simulink model "FSI_1DOF_Simscape"  (R2024a)
settings: Solver=FixedStepAuto  StartTime=0.0  StopTime=5  FixedStep=1e-4  MaxStep=1e-5  MinStep=1e-5  RelTol=1e-6  EnableMultiTasking=on
InitFcn:
  | FSI_1DOF_Simscape_init
values from neighbouring files (symbols this model uses):
  b = (2*m*omega_0)/(2*Q)    (= 3.14159265359)    [FSI_1DOF_Simscape_init.m]
  bias_exc = 0    [FSI_1DOF_Simscape_init.m]
  F_exc = 10    [FSI_1DOF_Simscape_init.m]
  omega_exc = 2*pi*freq_exc    (= 62.8318530718)    [FSI_1DOF_Simscape_init.m]
  phase_exc = 0    [FSI_1DOF_Simscape_init.m]
  t_step = 1e-2    (= 0.01)    [FSI_1DOF_Simscape_init.m]
libraries: fl_lib x8, nesl_utility x4
settings Model: Creator=FilipKsica  LastModifiedBy=144901
settings SolverCC: InitialStep=1e-5  AlgebraicLoopSolver=TrustRegion
settings DataIOCC: LimitDataPoints=on  ReturnWorkspaceOutputs=off
settings OptimizationCC: LifeSpan=inf
settings DebuggingCC: UnconnectedInputMsg=warning  UnconnectedOutputMsg=warning  UnconnectedLineMsg=warning  AllowSymbolicDim=off  SFUnexpectedBacktrackingDiag=warning  SFNoUnconditionalDefaultTransitionDiag=warning  SFExecutionAtInitializationDiag=none  ArithmeticOperatorsInVariantConditions=warning
settings ModelReferenceCC: EnableRefExpFcnMdlSchedulingChecks=on  PropagateSignalLabelsOutOfModel=off
settings SFSimCC: SimUseLocalCustomCode=off  CustomCodeUndefinedFunction=UseInterfaceOnly
settings RTWCC: RTWUseLocalCustomCode=off  GPUComputeCapability=3.5  DLArmComputeVersion=19.05
settings CodeAppCC: StateflowObjectComments=on
settings GRTTargetCC: TargetLangStandard=C89/C90 (ANSI)
settings ConfigComp: CovMetricSettings=dw  CovSaveCumulativeToWorkspaceVar=on  CovSaveSingleToWorkspaceVar=on  CovExternalEMLEnable=off
settings SimscapeCC: SimscapeNormalizeSystem=off

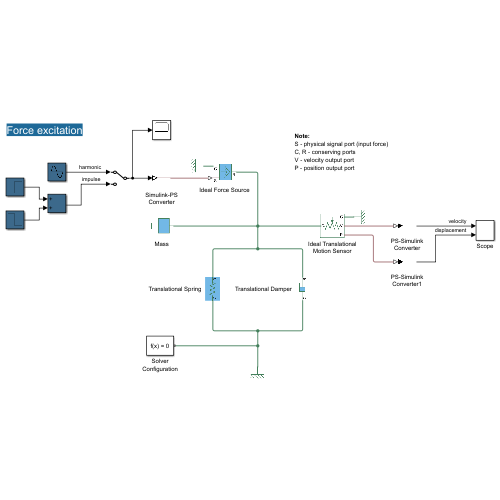
[thumbnail: Simulink's stored preview of the top-level diagram]
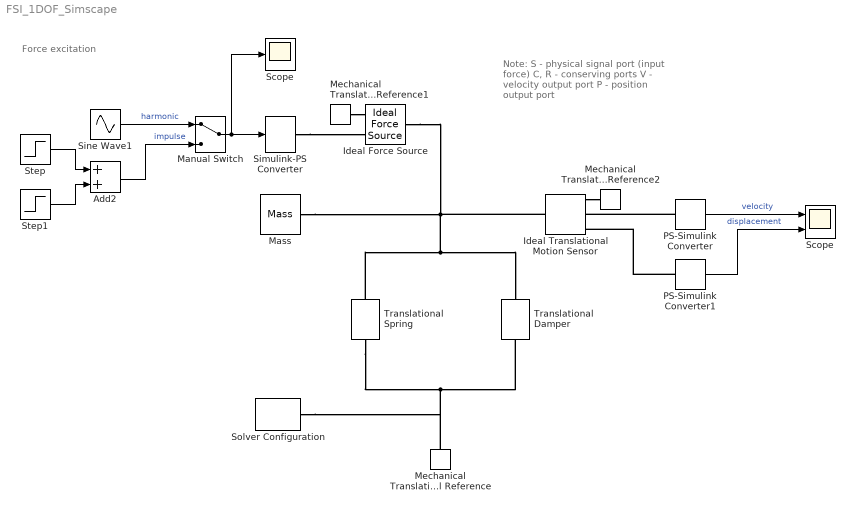
== system FSI_1DOF_Simscape ==
  note: Note:
      | S - physical signal port (input force)
      | C, R - conserving ports
      | V - velocity output port
      | P - position output port
  note: Force excitation
  Add2 : Sum
  Ideal Force Source : fl_lib/Mechanical/Mechanical Sources/Ideal Force Source
  Ideal Translational Motion Sensor : fl_lib/Mechanical/Mechanical Sensors/Ideal Translational Motion Sensor  reference=foundation.enum.MeasurementReference.difference  acceleration_port=false  velocity_port=true  position_port=true  offset=0 m
  Manual Switch : ManualSwitch
  Mass : fl_lib/Mechanical/Translational Elements/Mass  mass=m kg  num_ports=foundation.enum.numPorts2.one  v_specify=off  v_priority=None  v=0 m/s  v_nominal_specify=off  v_nominal_value=1  v_nominal_unit=m/s  f_specify=off  f_priority=None  f=0 N  f_nominal_specify=off  f_nominal_value=1  f_nominal_unit=N
  Mechanical Translational Reference : fl_lib/Mechanical/Translational Elements/Mechanical Translational Reference
  Mechanical Translational Reference1 : fl_lib/Mechanical/Translational Elements/Mechanical Translational Reference
  Mechanical Translational Reference2 : fl_lib/Mechanical/Translational Elements/Mechanical Translational Reference
  PS-Simulink Converter : nesl_utility/PS-Simulink Converter  PhysicalDomain=network_engine_domain  SubClassName=ps_output  LeftPortType=input  RightPortType=output  PseudoPeriodic=off  Frequencies=[]  VectorFormat=1-D array  Unit=1  AffineConversion=off
  PS-Simulink Converter1 : nesl_utility/PS-Simulink Converter  PhysicalDomain=network_engine_domain  SubClassName=ps_output  LeftPortType=input  RightPortType=output  PseudoPeriodic=off  Frequencies=[]  VectorFormat=1-D array  Unit=1  AffineConversion=off
  Scope : Scope
  "Scope " : Scope  NumInputPorts=2
  Simulink-PS Converter : nesl_utility/Simulink-PS Converter  PhysicalDomain=network_engine_domain  SubClassName=ps_input  LeftPortType=input  RightPortType=output  PseudoPeriodic=off  Frequencies=[]  NoiseDistribution=none  NoiseParameters=[]  Unit=1  AffineConversion=off  FilteringAndDerivatives=zero  SimscapeFilterOrder=1  InputFilterTimeConstant=0.001  UdotUserProvided=1
  Sine Wave1 : Sin  Amplitude=F_exc  Bias=bias_exc  Frequency=omega_exc  Phase=phase_exc  SampleTime=0
  Solver Configuration : nesl_utility/Solver Configuration  PhysicalDomain=network_engine_domain  SubClassName=solver  LeftPortType=input  RightPortType=generic  Tones=[]  Harmonics=[]  SimulateNoise=off  Profile=off  UseLocalSampling=off  EnableSwitchedLinearOptims=on  FrequencyDomain=off  UseCCode=off  RelTol=0.001  AbsTol=1e-06  MinStep=1e-09  ToWorkspace=off  RevertToSquareIcSolve=off  NumHomotopyIterations=100  PhasorMode=off  PhasorModeNumHarmonics=1  ConsistencySolver=NEWTON_FTOL  IndexReductionMethod=DerivativeReplacement  DoDC=off  ResidualTolerance=1e-09  ConsistencyTolSource=GLOBAL  ConsistencyAbsTol=0.001  ConsistencyRelTol=0.001  ConsistencyTolFactor=0.001  UseLocalSolver=off  LocalSolverChoice=NE_BACKWARD_EULER_ADVANCER  ResolveIndetEquations=on  FunctionEvalNumThread=1  LocalSolverSampleTime=0.001  DoFixedCost=off  MaxNonlinIter=3  MaxModeIter=2  ComputeImpulses=off  ImpulseIterations=2  LinearAlgebra=Sparse  LinearAlgebraNumThread=0  EquationFormulation=NE_TIME_EF  DelaysMemoryBudget=1024  AutomaticFiltering=on  FilteringTimeConstant=0.001  PartitionStorageMethod=AS_NEEDED  PartitionMemoryBudget=1024  PartitionMethod=FAST  MultibodyUseLocalSolver=off  MultibodyLocalSolverChoice=ODE1  MultibodyLocalSolverSampleTime=0.001
  Step : Step  Time=0  After=F_exc  SampleTime=0
  Step1 : Step  Time=t_step  After=-F_exc  SampleTime=0
  Translational Damper : fl_lib/Mechanical/Translational Elements/Translational Damper  D=b N/(m/s)  v_specify=off  v_priority=None  v=0 m/s  v_nominal_specify=off  v_nominal_value=1  v_nominal_unit=m/s  f_specify=off  f_priority=None  f=0 N  f_nominal_specify=off  f_nominal_value=1  f_nominal_unit=N
  Translational Spring : fl_lib/Mechanical/Translational Elements/Translational Spring  spr_rate=k N/m  v_specify=off  v_priority=None  v=0 m/s  v_nominal_specify=off  v_nominal_value=1  v_nominal_unit=m/s  f_specify=off  f_priority=None  f=0 N  f_nominal_specify=off  f_nominal_value=1  f_nominal_unit=N  x_specify=off  x_priority=None  x=0 m  x_nominal_specify=off  x_nominal_value=1  x_nominal_unit=m
  wires:
  PS-Simulink Converter/1 -> "Scope "/1  "velocity"
  Step/1 -> Add2/1
  Step1/1 -> Add2/2
  Manual Switch/1 -> Simulink-PS Converter/1, Scope/1
  Sine Wave1/1 -> Manual Switch/1  "harmonic"
  Add2/1 -> Manual Switch/2  "impulse"
  PS-Simulink Converter1/1 -> "Scope "/2  "displacement"
  connections:
  Mechanical Translational Reference1/LConn1 -- Ideal Force Source/RConn2
  Translational Spring/LConn1 -- Translational Damper/LConn1 -- Ideal Translational Motion Sensor/LConn1 -- Ideal Force Source/LConn1 -- Mass/LConn1
  Translational Spring/RConn1 -- Mechanical Translational Reference/LConn1 -- Solver Configuration/RConn1 -- Translational Damper/RConn1
  PS-Simulink Converter1/LConn1 -- Ideal Translational Motion Sensor/RConn3
  PS-Simulink Converter/LConn1 -- Ideal Translational Motion Sensor/RConn2
  Simulink-PS Converter/RConn1 -- Ideal Force Source/RConn1
  Ideal Translational Motion Sensor/RConn1 -- Mechanical Translational Reference2/LConn1
